simulink model "main"  (R2023a)
settings: Solver=VariableStepAuto  StartTime=0.0  StopTime=inf  RelTol=1e-3
libraries: Visualization x1, DataAcquisition x1
settings Model: Creator=circuit  LastModifiedBy=circuit

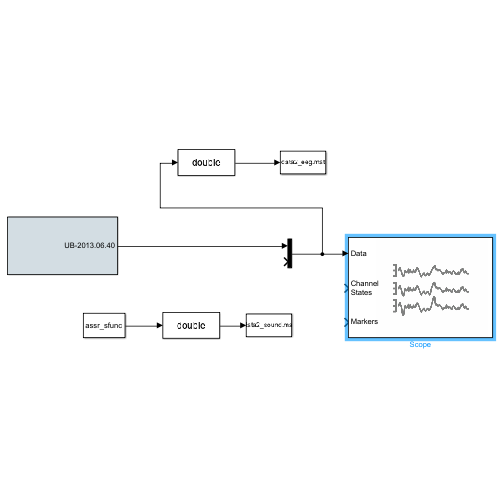
[thumbnail: Simulink's stored preview of the top-level diagram]
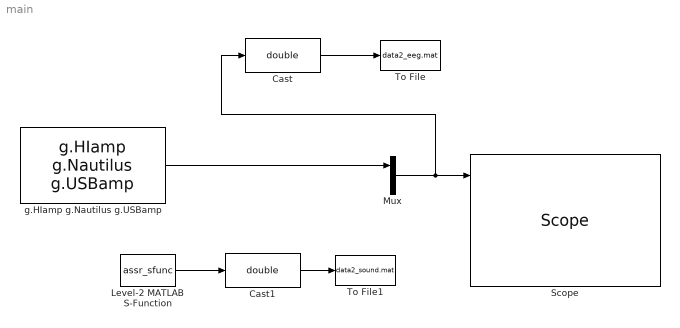
== system main ==
  Cast : DataTypeConversion  OutDataTypeStr=double  SaturateOnIntegerOverflow=off  RndMeth=Floor
  Cast1 : DataTypeConversion  OutDataTypeStr=double  SaturateOnIntegerOverflow=off  RndMeth=Floor
  Level-2 MATLAB S-Function : M-S-Function  FunctionName=assr_sfunc
  Mux : Mux  Inputs=2
  Scope : Visualization/Scope
      settings: SourceProductName=g.HIsys
  To File : ToFile  Filename=data2_eeg.mat  MatrixName=Y
  To File1 : ToFile  Filename=data2_sound.mat  MatrixName=Y
  g.HIamp g.Nautilus g.USBamp : DataAcquisition/g.HIamp g.Nautilus g.USBamp  cfgUpdated=739913.438  numDevices=2  deviceSR=[500 250 ]  deviceChannels=[9 4 ]  numSR=[2 ]  SRIndexPerDevice=[1 0 ]
      settings: SourceProductName=g.HIsys
  wires:
  g.HIamp g.Nautilus g.USBamp/1 -> Mux/1
  Mux/1 -> Cast/1, Scope/1
  Cast/1 -> To File/1
  Level-2 MATLAB S-Function/1 -> Cast1/1
  Cast1/1 -> To File1/1
